simulink model "tilting_control_voliro_template"  (R2024b)
settings: Solver=VariableStepAuto  StartTime=0.0  StopTime=30  RelTol=1e-3
InitFcn:
  | %% INITIALIZATION
  | 
  | %% UAV PARAMETERS
  | 
  | mass = 1.32;
  | Ib = diag([0.0154 0.0154 0.0263]);
  | cf = 1.65776*10^(-5);
  | cm = 2.1792*10^(-7);
  | l = 0.45;
  | 
  | %% SAMPLING TIME
  | Ts=0.001;
  | 
  | %% PLANNER
  | t_iniz = 0;
  | ttot=20; %duration
  | tdead=10; %dead time to evaluate the steady-state
  | tot_time = ttot + tdead;
  | t1=linspace(0,ttot,round(ttot/Ts));
  | t=linspace(0,ttot+tdead,round(ttot/Ts)+round(tdead/Ts));
  | p= zeros(4,length(t1)); dot_p= zeros(4,length(t1)); ddot_p= zeros(4,length(t1));
  | p_d= zeros(4,length(t)); dot_p_d= zeros(4,length(t)); ddot_p_d= zeros(4,length(t));
  | Rbdes = zeros(3,3,length(t));
  | omegabb_des = zeros(3,length(t));
  | dot_omegabb_des = zeros(3,length(t));
  | 
  | %Initial and final conditions
  | x0= 0; xf=1; dot_x0= 0; dot_xf=0; ddot_x0=0; ddot_xf=0; dddot_x0 = 0; dddot_xf = 0;
  | y0= 0; yf=1; dot_y0= 0; dot_yf=0; ddot_y0=0; ddot_yf=0; dddot_y0 = 0; dddot_yf = 0;
  | z0= -1; zf=-4; dot_z0= 0; dot_zf=0; ddot_z0=0; ddot_zf=0; dddot_z0 = 0; dddot_zf = 0;
  | Rb0 = eye(3);
  | roll_f = pi/4; pitch_f = pi/4; yaw_f = pi;%radians
  | Rf = [cos(pitch_f)*cos(yaw_f) sin(roll_f)*sin(pitch_f)*cos(yaw_f)-cos(roll_f)*sin(yaw_f) cos(roll_f)*sin(pitch_f)*cos(yaw_f)+sin(roll_f)*sin(yaw_f);
  |     cos(pitch_f)*sin(yaw_f) sin(roll_f)*sin(pitch_f)*sin(yaw_f)+cos(roll_f)*cos(yaw_f) cos(roll_f)*sin(pitch_f)*sin(yaw_f)-sin(roll_f)*cos(yaw_f);
  |     -sin(pitch_f) sin(roll_f)*cos(pitch_f) cos(roll_f)*cos(pitch_f)];
  | Rbf = Rb0'*Rf;
  | theta_f = acos(0.5*(Rbf(1,1)+Rbf(2,2)+Rbf(3,3)-1));
  | axis_r = (1/2/sin(theta_f))*[Rbf(3,2)-Rbf(2,3);Rbf(1,3)-Rbf(3,1);Rbf(2,1)-Rbf(1,2)];
  | theta_0 = 0;
  | 
  | p0=[x0,y0,z0,theta_0]; dot_p0=[dot_x0,dot_y0,dot_z0,0]; ddot_p0=[ddot_x0,ddot_y0,ddot_z0,0]; dddot_p0=[dddot_x0,dddot_y0,dddot_z0,0];
  | pf=[xf,yf,zf,theta_f]; dot_pf=[dot_xf,dot_yf,dot_zf,0]; ddot_pf=[ddot_xf,ddot_yf,ddot_zf,0]; dddot_pf=[dddot_xf,dddot_yf,dddot_zf,0];
  | %7-th order polynomial
  | a0=zeros(1,4); a1=zeros(1,4); a2=zeros(1,4); a3=zeros(1,4); a4=zeros(1,4); a5=zeros(1,4); a6 = zeros(1,4); a7 = zeros(1,4);
  | 
  | for j=1:4
  |     A = [t_iniz^7, t_iniz^6, t_iniz^5, t_iniz^4, t_iniz^3, t_iniz^2, t_iniz, 1;
  |         ttot^7, ttot^6, ttot^5, ttot^4, ttot^3, ttot^2, ttot, 1;
  |         7*t_iniz^6, 6*t_iniz^5, 5*t_iniz^4, 4*t_iniz^3, 3*t_iniz^2, 2*t_iniz, 1, 0;
  |         7*ttot^6, 6*ttot^5, 5*ttot^4, 4*ttot^3, 3*ttot^2, 2*ttot, 1, 0;
  |         42*t_iniz^5, 30*t_iniz^4, 20*t_iniz^3, 12*t_iniz^2, 6*t_iniz, 2, 0, 0;
  |         42*ttot^5, 30*ttot^4, 20*ttot^3, 12*ttot^2, 6*ttot, 2, 0, 0;
  |         210*t_iniz^4, 120*t_iniz^3, 60*t_iniz^2, 24*t_iniz, 6, 0, 0, 0;
  |         210*ttot^4, 120*ttot^3, 60*ttot^2, 24*ttot, 6, 0, 0, 0];
  |     b = [p0(j) pf(j) dot_p0(j) dot_pf(j) ddot_p0(j) ddot_pf(j) dddot_p0(j) dddot_pf(j)]';
  |     a_temp = A\b;
  |     a7(j) = a_temp(1);
  |     a6(j) = a_temp(2);
  |     a5(j) = a_temp(3);
  |     a4(j) = a_temp(4);
  |     a3(j) = a_temp(5);
  |     a2(j) = a_temp(6);
  |     a1(j) = a_temp(7);
  |     a0(j) = a_temp(8);
  | 
  |     %trajectories
  |     p(j,:)=a7(j)*t1.^7 + a6(j)*t1.^6 + a5(j)*t1.^5 +a4(j)*t1.^4 +a3(j)*t1.^3 +a2(j)*t1.^2 +a1(j)*t1 +a0(j);
  |     dot_p(j,:) = 7*a7(j)*t1.^6 + 6*a6(j)*t1.^5 + 5*a5(j)*t1.^4 +4*a4(j)*t1.^3 +3*a3(j)*t1.^2 +2*a2(j)*t1 +a1(j);
  |     ddot_p(j,:) = 42*a7(j)*t1.^5 + 30*a6(j)*t1.^4 + 20*a5(j)*t1.^3 + 12*a4(j)*t1.^2 + 6*a3(j)*t1 +2*a2(j);
  |     dddot_p(j,:) = 210*a7(j)*t1.^4 + 120*a6(j)*t1.^3 + 60*a5(j)*t1.^2 + 24*a4(j)*t1 + 6*a3(j);
  |     %addition of the stead-state terms
  |     p_d(j,:)=[p(j,:) zeros(1,round(tdead/Ts))+pf(j)];
  |     dot_p_d(j,:)=[dot_p(j,:) zeros(1,round(tdead/Ts))+dot_pf(j)];
  |     ddot_p_d(j,:)=[ddot_p(j,:) zeros(1,round(tdead/Ts))+ddot_pf(j)];
  |     dddot_p_d(j,:)=[dddot_p(j,:) zeros(1,round(tdead/Ts))+dddot_pf(j)];
  | end
  | for i = 1:length(t)
  |     tetai = p_d(4,i);
  |     dot_tetai = dot_p_d(4,i);
  |     ddot_tetai = ddot_p_d(4,i);
  |     temp1 = 1-cos(tetai);
  |     Ri = [axis_r(1)^2*temp1+cos(tetai) axis_r(1)*axis_r(2)*temp1-axis_r(3)*sin(tetai) axis_r(1)*axis_r(3)*temp1+axis_r(2)*sin(tetai);
  |         axis_r(1)*axis_r(2)*temp1+axis_r(3)*sin(tetai) axis_r(2)^2*temp1+cos(tetai) axis_r(2)*axis_r(3)*temp1-axis_r(1)*sin(tetai);
  |         axis_r(1)*axis_r(3)*temp1-axis_r(2)*sin(tetai) axis_r(2)*axis_r(3)*temp1+axis_r(1)*sin(tetai) axis_r(3)^2*temp1+cos(tetai)];
  |     Rbdes(:,:,i) = Rb0*Ri;
  |     omegabb_des(:,i) = Rbdes(:,:,i)'*Rb0*axis_r*dot_tetai;
  |     dot_omegabb_des(:,i) = Rbdes(:,:,i)'*Rb0*axis_r*ddot_tetai;
  | end
  | %data for Simulink
  | pos_0 = [x0 y0 z0];
  | lin_vel_0 = [dot_x0 dot_y0 dot_z0];
  | w_bb_0 = [0 0 0];
  | csi_d=p_d(1:3,:); dot_csi_d=dot_p_d(1:3,:); ddot_csi_d=ddot_p_d(1:3,:); dddot_csi_d = dddot_p_d(1:3,:);
  | psi_d=p_d(4,:); dot_psi_d=dot_p_d(4,:); ddot_psi_d=ddot_p_d(4,:); dddot_psi_d = dddot_p_d(4,:);
libraries: robotcorelib x1, matrix_library x1, uavutilslib x1
settings Model: Creator=fabioruggiero  LastModifiedBy=feder
settings ModelReferenceCC: EnableRefExpFcnMdlSchedulingChecks=on
settings RTWCC: GPUComputeCapability=3.5

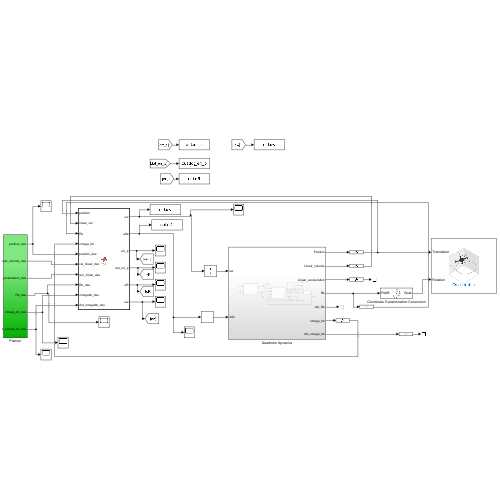
[thumbnail: Simulink's stored preview of the top-level diagram]
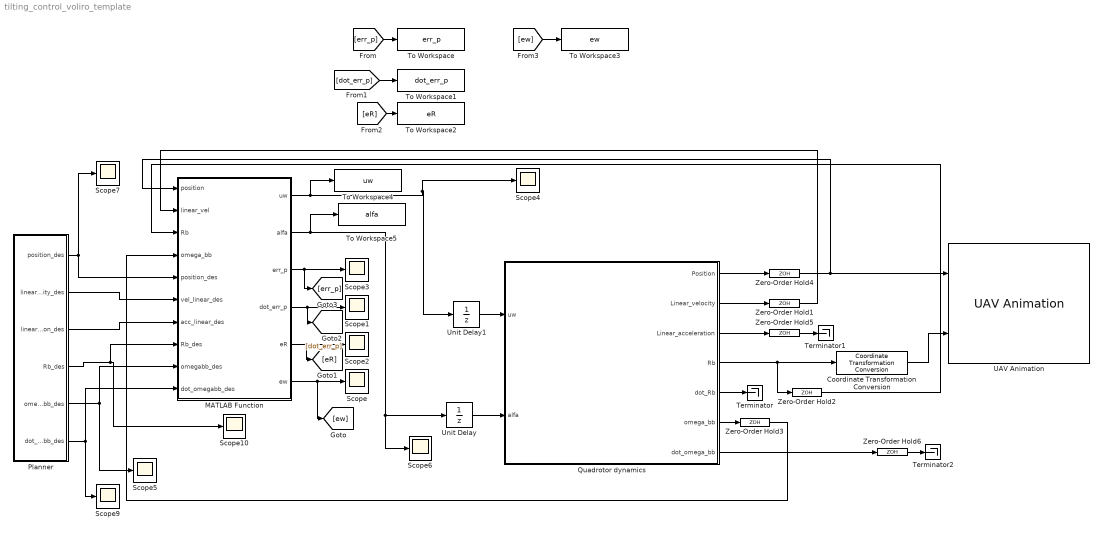
== system tilting_control_voliro_template ==
  Coordinate Transformation Conversion : robotcorelib/Coordinate Transformation Conversion  InputRepresentation=Rotation Matrix  InputEulerSequence=ZYX  ShowTrVecInputPort=on  OutputRepresentation=Quaternion  OutputEulerSequence=ZYX  ShowTrVecOutputPort=on  SimulateUsing=Interpreted execution
  MATLAB Function : MATLAB Function  TreatAsAtomicUnit=on
  Planner : Subsystem
  Quadrotor dynamics : Subsystem
  Scope{,1..7,9..10} (10 alike) : Scope
  Terminator : Terminator
  Terminator1 : Terminator
  Terminator2 : Terminator
  To Workspace : ToWorkspace  VariableName=err_p  SaveFormat=Timeseries  SampleTime=-1
  To Workspace1 : ToWorkspace  VariableName=dot_err_p  SaveFormat=Timeseries  SampleTime=-1
  To Workspace2 : ToWorkspace  VariableName=eR  SaveFormat=Timeseries  SampleTime=-1
  To Workspace3 : ToWorkspace  VariableName=ew  SaveFormat=Timeseries  SampleTime=-1
  To Workspace4 : ToWorkspace  VariableName=uw  SaveFormat=Timeseries  SampleTime=-1
  To Workspace5 : ToWorkspace  VariableName=alfa  SaveFormat=Timeseries  SampleTime=-1
  UAV Animation : uavutilslib/UAV Animation  NumUAV=1  DynamicUAVConfig=off  UAVType=Multirotor  UAVSize=1  UAVColor=[1 0 0]  UAVTrajectoryAlpha=1  InertialZDirection=Down  RotationFormat=Quaternion  DrawMarkers=off  SampleTime=0.01
  Unit Delay : UnitDelay  InitialCondition=[0; 0; 0; 0]  SampleTime=-1  HasFrameUpgradeWarning=on
  Unit Delay1 : UnitDelay  InitialCondition=1.952815847891130e+05*ones(4,1)  SampleTime=-1  HasFrameUpgradeWarning=on
  Zero-Order Hold{1..6} (6 alike) : ZeroOrderHold  SampleTime=Ts
  wires:
  MATLAB Function/1(uw) -> To Workspace4/1, Scope4/1, Unit Delay1/1
  Quadrotor dynamics/1(Position) -> Zero-Order Hold4/1
  Quadrotor dynamics/2(Linear_velocity) -> Zero-Order Hold1/1
  Quadrotor dynamics/4(Rb) -> Zero-Order Hold2/1, Coordinate Transformation Conversion/1
  Quadrotor dynamics/6(omega_bb) -> Zero-Order Hold3/1
  Zero-Order Hold4/1 -> MATLAB Function/1(position), UAV Animation/1
  Quadrotor dynamics/5(dot_Rb) -> Terminator/1
  Planner/1(position_des) -> Scope7/1, MATLAB Function/5(position_des)
  Planner/2(linear_velocity_des) -> MATLAB Function/6(vel_linear_des)
  Coordinate Transformation Conversion/1 -> UAV Animation/2
  MATLAB Function/6(ew) -> [ew], Scope/1
  MATLAB Function/4(dot_err_p) -> [dot_err_p], Scope1/1
  Quadrotor dynamics/3(Linear_acceleration) -> Zero-Order Hold5/1
  Planner/3(linear_acceleration_des) -> MATLAB Function/7(acc_linear_des)
  MATLAB Function/5(eR) -> [eR], Scope2/1
  MATLAB Function/3(err_p) -> [err_p], Scope3/1
  Zero-Order Hold1/1 -> MATLAB Function/2(linear_vel)
  Zero-Order Hold2/1 -> MATLAB Function/3(Rb)
  Zero-Order Hold3/1 -> MATLAB Function/4(omega_bb)
  Quadrotor dynamics/7(dot_omega_bb) -> Zero-Order Hold6/1
  MATLAB Function/2(alfa) -> To Workspace5/1, Scope6/1, Unit Delay/1
  Unit Delay/1 -> Quadrotor dynamics/2(alfa)
  Unit Delay1/1 -> Quadrotor dynamics/1(uw)
  Planner/4(Rb_des) -> Scope10/1, MATLAB Function/8(Rb_des)
  Planner/5(omega_bb_des) -> MATLAB Function/9(omegabb_des), Scope5/1
  Planner/6(dot_omega_bb_des) -> MATLAB Function/10(dot_omegabb_des), Scope9/1
  Zero-Order Hold5/1 -> Terminator1/1
  Zero-Order Hold6/1 -> Terminator2/1
  [err_p] -> To Workspace/1
  [dot_err_p] -> To Workspace1/1
  [eR] -> To Workspace2/1
  [ew] -> To Workspace3/1

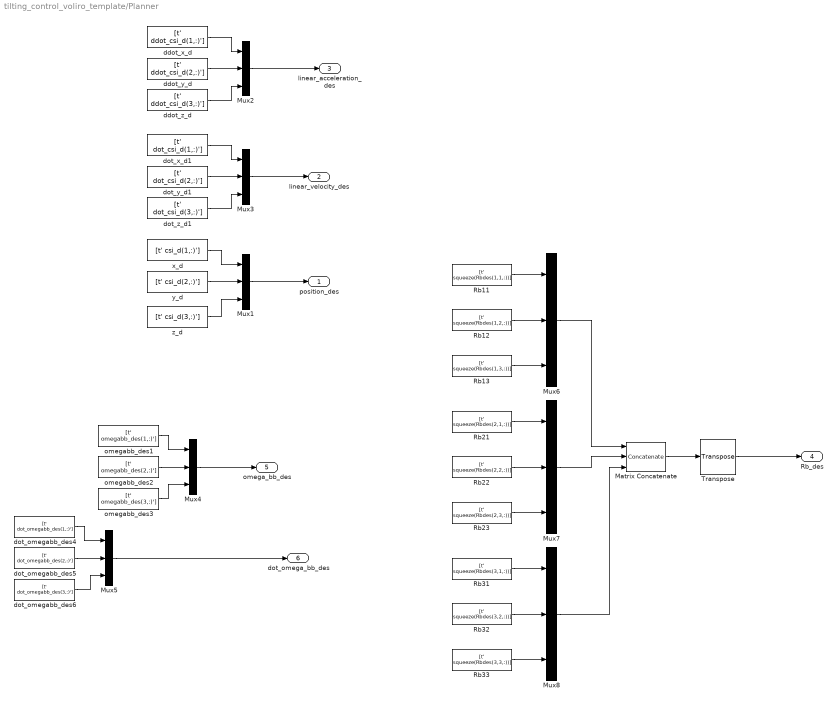
== system tilting_control_voliro_template/Planner ==
  Matrix Concatenate : Concatenate  NumInputs=3  Mode=Multidimensional array  ConcatenateDimension=2
  Mux{1..8} (8 alike) : Mux  Inputs=3
  Rb11 : FromWorkspace  VariableName=[t' squeeze(Rbdes(1,1,:))]  SampleTime=Ts
  Rb12 : FromWorkspace  VariableName=[t' squeeze(Rbdes(1,2,:))]  SampleTime=Ts
  Rb13 : FromWorkspace  VariableName=[t' squeeze(Rbdes(1,3,:))]  SampleTime=Ts
  Rb21 : FromWorkspace  VariableName=[t' squeeze(Rbdes(2,1,:))]  SampleTime=Ts
  Rb22 : FromWorkspace  VariableName=[t' squeeze(Rbdes(2,2,:))]  SampleTime=Ts
  Rb23 : FromWorkspace  VariableName=[t' squeeze(Rbdes(2,3,:))]  SampleTime=Ts
  Rb31 : FromWorkspace  VariableName=[t' squeeze(Rbdes(3,1,:))]  SampleTime=Ts
  Rb32 : FromWorkspace  VariableName=[t' squeeze(Rbdes(3,2,:))]  SampleTime=Ts
  Rb33 : FromWorkspace  VariableName=[t' squeeze(Rbdes(3,3,:))]  SampleTime=Ts
  Transpose : matrix_library/Transpose
  ddot_x_d : FromWorkspace  VariableName=[t' ddot_csi_d(1,:)']  SampleTime=Ts
  ddot_y_d : FromWorkspace  VariableName=[t' ddot_csi_d(2,:)']  SampleTime=Ts
  ddot_z_d : FromWorkspace  VariableName=[t' ddot_csi_d(3,:)']  SampleTime=Ts
  dot_omegabb_des4 : FromWorkspace  VariableName=[t' dot_omegabb_des(1,:)']  SampleTime=Ts
  dot_omegabb_des5 : FromWorkspace  VariableName=[t' dot_omegabb_des(2,:)']  SampleTime=Ts
  dot_omegabb_des6 : FromWorkspace  VariableName=[t' dot_omegabb_des(3,:)']  SampleTime=Ts
  dot_x_d1 : FromWorkspace  VariableName=[t' dot_csi_d(1,:)']  SampleTime=Ts
  dot_y_d1 : FromWorkspace  VariableName=[t' dot_csi_d(2,:)']  SampleTime=Ts
  dot_z_d1 : FromWorkspace  VariableName=[t' dot_csi_d(3,:)']  SampleTime=Ts
  omegabb_des1 : FromWorkspace  VariableName=[t' omegabb_des(1,:)']  SampleTime=Ts
  omegabb_des2 : FromWorkspace  VariableName=[t' omegabb_des(2,:)']  SampleTime=Ts
  omegabb_des3 : FromWorkspace  VariableName=[t' omegabb_des(3,:)']  SampleTime=Ts
  x_d : FromWorkspace  VariableName=[t' csi_d(1,:)']  SampleTime=Ts
  y_d : FromWorkspace  VariableName=[t' csi_d(2,:)']  SampleTime=Ts
  z_d : FromWorkspace  VariableName=[t' csi_d(3,:)']  SampleTime=Ts
  position_des : Outport
  linear_velocity_des : Outport  Port=2
  linear_acceleration_des : Outport  Port=3
  Rb_des : Outport  Port=4
  omega_bb_des : Outport  Port=5
  dot_omega_bb_des : Outport  Port=6
  wires:
  y_d/1 -> Mux1/2
  z_d/1 -> Mux1/3
  x_d/1 -> Mux1/1
  ddot_y_d/1 -> Mux2/2
  ddot_z_d/1 -> Mux2/3
  ddot_x_d/1 -> Mux2/1
  Mux2/1 -> linear_acceleration_des/1
  Mux1/1 -> position_des/1
  dot_y_d1/1 -> Mux3/2
  dot_z_d1/1 -> Mux3/3
  dot_x_d1/1 -> Mux3/1
  Mux3/1 -> linear_velocity_des/1
  Mux5/1 -> dot_omega_bb_des/1
  omegabb_des3/1 -> Mux4/3
  Mux4/1 -> omega_bb_des/1
  omegabb_des2/1 -> Mux4/2
  omegabb_des1/1 -> Mux4/1
  dot_omegabb_des4/1 -> Mux5/1
  dot_omegabb_des5/1 -> Mux5/2
  dot_omegabb_des6/1 -> Mux5/3
  Rb11/1 -> Mux6/1
  Rb12/1 -> Mux6/2
  Rb13/1 -> Mux6/3
  Rb23/1 -> Mux7/3
  Rb22/1 -> Mux7/2
  Rb21/1 -> Mux7/1
  Rb31/1 -> Mux8/1
  Rb32/1 -> Mux8/2
  Rb33/1 -> Mux8/3
  Mux6/1 -> Matrix Concatenate/1
  Mux7/1 -> Matrix Concatenate/2
  Mux8/1 -> Matrix Concatenate/3
  Matrix Concatenate/1 -> Transpose/1
  Transpose/1 -> Rb_des/1

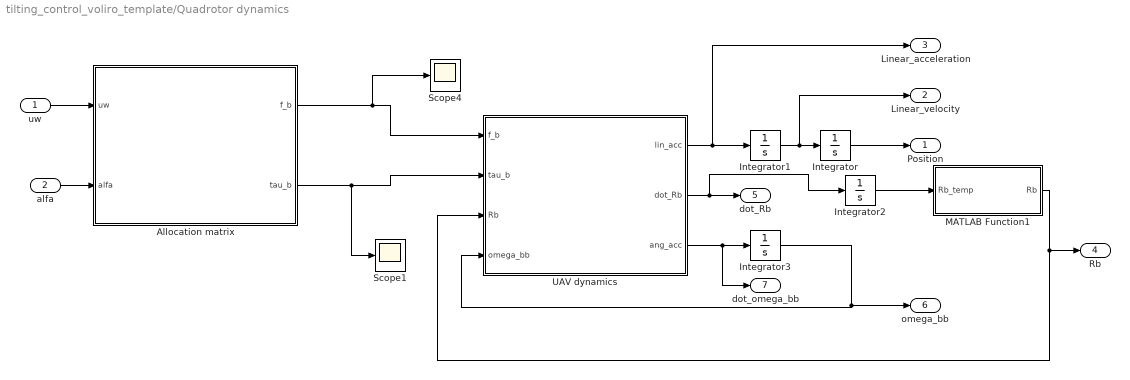
== system tilting_control_voliro_template/Quadrotor dynamics ==
  uw : Inport
  alfa : Inport  Port=2
  Allocation matrix : MATLAB Function  TreatAsAtomicUnit=on
  Integrator : Integrator  InitialCondition=pos_0
  Integrator1 : Integrator  InitialCondition=lin_vel_0
  Integrator2 : Integrator  InitialCondition=[1 0 0; 0 1 0;0 0 1]
  Integrator3 : Integrator  InitialCondition=w_bb_0
  MATLAB Function1 : MATLAB Function  TreatAsAtomicUnit=on
  Scope1 : Scope
  Scope4 : Scope
  UAV dynamics : MATLAB Function  TreatAsAtomicUnit=on
  Position : Outport
  Linear_velocity : Outport  Port=2
  Linear_acceleration : Outport  Port=3
  Rb : Outport  Port=4
  dot_Rb : Outport  Port=5
  omega_bb : Outport  Port=6
  dot_omega_bb : Outport  Port=7
  wires:
  Integrator/1 -> Position/1
  UAV dynamics/3(ang_acc) -> dot_omega_bb/1, Integrator3/1
  Integrator1/1 -> Linear_velocity/1, Integrator/1
  Integrator3/1 -> UAV dynamics/4(omega_bb), omega_bb/1
  UAV dynamics/2(dot_Rb) -> Integrator2/1, dot_Rb/1
  MATLAB Function1/1(Rb) -> Rb/1, UAV dynamics/3(Rb)
  Integrator2/1 -> MATLAB Function1/1(Rb_temp)
  uw/1 -> Allocation matrix/1(uw)
  alfa/1 -> Allocation matrix/2(alfa)
  Allocation matrix/1(f_b) -> Scope4/1, UAV dynamics/1(f_b)
  UAV dynamics/1(lin_acc) -> Linear_acceleration/1, Integrator1/1
  Allocation matrix/2(tau_b) -> Scope1/1, UAV dynamics/2(tau_b)

== matlab function tilting_control_voliro_template/Quadrotor dynamics/Allocation matrix ==
  data: uw input size=4; alfa input size=4; f_b output size=3; tau_b output size=3; cm parameter; cf parameter; l parameter
function [f_b,tau_b] = fcn(uw,alfa,cm, cf, l)

alfa1 = alfa(1);
alfa2 = alfa(2);
alfa3 = alfa(3);
alfa4 = alfa(4);


Gq = [0 -cf*sin(alfa2) 0 cf*sin(alfa4);
    cf*sin(alfa1) 0 -cf*sin(alfa3) 0;
    -cf*cos(alfa1) -cf*cos(alfa2) -cf*cos(alfa3) -cf*cos(alfa4);
    0 -l*cf*cos(alfa2)-cm*sin(alfa2) 0 l*cf*cos(alfa4)+cm*sin(alfa4);
    l*cf*cos(alfa1)+cm*sin(alfa1) 0 -l*cf*cos(alfa3)-cm*sin(alfa3) 0;
    l*cf*sin(alfa1)-cm*cos(alfa1) -l*cf*sin(alfa2)+cm*cos(alfa2) l*cf*sin(alfa3)-cm*cos(alfa3) -l*cf*sin(alfa4)+cm*cos(alfa4)];
out = Gq*uw;
f_b = out(1:3);
tau_b = out(4:6);
end

== matlab function tilting_control_voliro_template/Quadrotor dynamics/UAV dynamics ==
  data: f_b input size=3; tau_b input size=3; lin_acc output size=3; Rb input size=[3,3]; omega_bb input size=3; dot_Rb output size=[3,3]; ang_acc output size=3; mass parameter size=1; Ib parameter size=[3,3]
function [lin_acc, dot_Rb, ang_acc] = fcn(f_b,tau_b,Rb,omega_bb,mass, Ib)

lin_acc = 9.81*[0 0 1]'+(1/mass)*Rb*f_b;
dot_Rb = Rb*skew(omega_bb);
ang_acc = inv(Ib)*(-skew(omega_bb)*Ib*omega_bb + tau_b);

end

function S = skew(v)
if(numel(v)~= 1)
S= [0 -v(3) v(2); 
    v(3) 0 -v(1);
    -v(2) v(1) 0];
else
S= zeros(3);
end
end

== matlab function tilting_control_voliro_template/MATLAB Function ==
  data: position input size=3; uw output size=4; linear_vel input size=3; Rb input size=[3,3]; omega_bb input size=3; position_des input size=3; vel_linear_des input size=3; acc_linear_des input size=3; Rb_des input size=[3,3]; omegabb_des input; dot_omegabb_des input; alfa output size=4; err_p output size=3; dot_err_p output size=3; eR output size=3; cf parameter; cm parameter; ew output size=3; mass parameter; Ib parameter; l parameter
function [uw,alfa, err_p, dot_err_p, eR, ew] = fcn(position, linear_vel, Rb, omega_bb, position_des, vel_linear_des, acc_linear_des, Rb_des, omegabb_des, dot_omegabb_des, cf, cm, mass, Ib, l)

%% WRITE HERE THE CONTROL FOR THE TILTING PROPELLER UAV
% position: linear position measure
% linear_vel: linear velocity measure
% Rb: current rotation matrix
% omega_bb: current angular velocity in the body frame
% positon_des: desired linear position from the planner
% vel_linear_des: desired linear velocity from the planner
% acc_linear_des: desired linear acceleration from the planner
% Rb_des: desired rotation matrix
% omega_des: desired angular velocity
% dot_omega_des: desired angular acceleration
% cf: thrust coefficient of the UAV
% cm: drag coefficient of the UAV
% mass: mass of the UAV
% Ib: inertia of the UAV
% l: distance between the propellers and the UAV's CoM
% ---
% uw: spinning propellers velocity
% alfa: tilting angle command
% err_p: position error
% dot_err_p: time derivative of the positon error
% eR: rotation matrix error
% ew: angular velocity error

 
  g  = 9.81;
  e3 = [0 0 1]';

  K_P=diag([6, 6, 8]);
  K_V=diag([4, 4, 5]);
  K_R=diag([3, 3, 3]);
  K_W=diag([4, 4, 4]);

  err_p     = position   - position_des;      
  dot_err_p = linear_vel - vel_linear_des;    
  eR = 0.5*vee( Rb_des'*Rb - Rb'*Rb_des );                
  ew = omega_bb - Rb' * Rb_des * omegabb_des;  

  M_bar=[mass*eye(3) zeros(3); zeros(3) Ib];
  g_bar=[mass*g*e3; -skew(omega_bb)*Ib*omega_bb];
  % b=inv(M_bar)*g_bar;
  b = M_bar \ g_bar;
  Matrix=[Rb zeros(3); zeros(3) eye(3)];

  G = [
      0    0    0    -1   0    0    0    1;   
      0    1    0    0    0   -1    0    0;   
     -1    0   -1    0   -1    0   -1    0;   
      0    0   -l  -cm/cf   0    0    l  cm/cf; 
      l cm/cf   0    0   -l -cm/cf   0  0; 
   -cm/cf  l  cm/cf  -l -cm/cf   l cm/cf   -l  
  ];


  A=pinv(M_bar)*Matrix*G;

  acc_linear=-K_P*err_p-K_V*dot_err_p+acc_linear_des;
  dot_omegabb= -K_R*eR-K_W*ew+dot_omegabb_des;

  %V=[acc_linear_des; dot_omegabb_des];
  v=[acc_linear; dot_omegabb];
  u=pinv(A)*(-b+v);
  %u=pinv(A)*(-b+V);
  % u_v=[u(1);u(3);u(5);u(7)];
  % u_l=[u(2);u(4);u(6);u(8)];
  u_v = u(1:2:end, :);  
  u_l = u(2:2:end, :);  
  
  uw   = zeros(4,1); %ok
  alfa = zeros(4,1); %ok

  for i = 1:4
    uw(i)   = (1/cf)*sqrt(u_v(i)^2 + u_l(i)^2);
    alfa(i) = atan2(u_l(i), u_v(i));
  end

 

end


function S = skew(v)
if(numel(v)~= 1)
S= [0 -v(3) v(2); 
    v(3) 0 -v(1);
    -v(2) v(1) 0];
else
S= zeros(3);
end
end

function v = vee(S)
v = [S(3,2); S(1,3); S(2,1)];
end

== matlab function tilting_control_voliro_template/Quadrotor dynamics/MATLAB Function1 ==
  data: Rb_temp input; Rb output
function Rb = fcn(Rb_temp)
    [U,S,V] = svd(Rb_temp);
    sigma = det(U*V');
    S_ = diag([1 1 sigma]);

    Rb = U*S_*V';
end
